simulink model "bmsTestPlatform"  (R2025b)
settings: configuration reference "cfgHarness" (kept outside this file)
PreLoadFcn:
  | if isempty(matlab.project.rootProject)
  |     % Opened outside the project (e.g. by RT-LAB): open it, then return to this folder
  |     d = pwd;
  |     try, openProject(fullfile(d, "..")); catch e, warning(e.message); end
  |     cd(d);
  | end
InitFcn:
  | plant_params
  | sensor_params
  | load_params
undefined symbols (not defined in the file): ADV_tStale, ARB_socTol, batMod, battery_builder_rtmsupport, BMS_state, BMS_stubOut, CAN_Ts, DiscIntNeverNeededParam, f, gcbh, HW_nvm, HW_powerPress, HW_resetPress, HW_rtcStart, LOAD_cycleA, LOAD_cycleAext, LOAD_iConst, LOAD_iPulse, LOAD_profile, LOAD_pulseDuty, LOAD_pulsePeriod, LOAD_scale, PLANT_switchFault, PLANT_tAmbient, PLANT_tContactor, PLANT_Ts, sens, SENS_faultChannel, SENS_faultDuration, SENS_faultRamp, SENS_faultStart, SENS_faultType, SENS_faultValue, SOC0, T0
libraries: bat_13S7P_detailed_lib x7, fl_lib x5, nesl_utility x4, simulink x3, instrumentlib x2
(part 1 of 2)
settings Model: DataDictionary=bmsPlatform.sldd  Creator=SC-Br  LastModifiedBy=SC-Br
settings ConfigSetRef: SourceName=cfgHarness

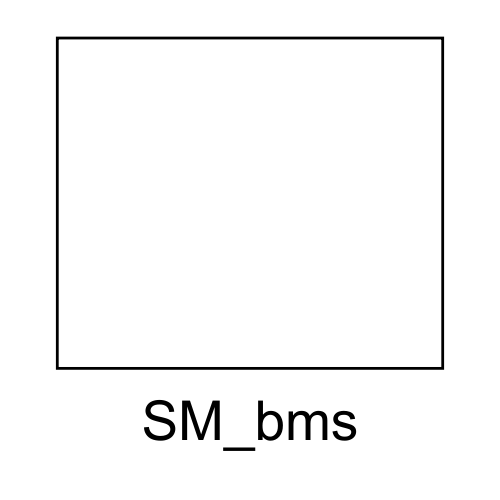
[thumbnail: Simulink's stored preview of the top-level diagram]
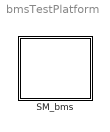
== system bmsTestPlatform ==
  SM_bms : Subsystem

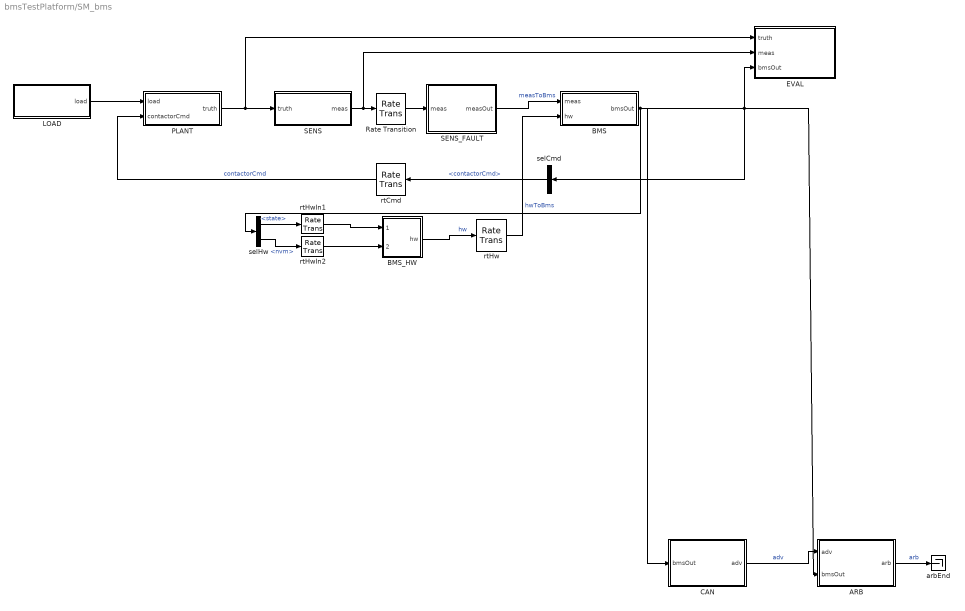
== system bmsTestPlatform/SM_bms ==
  ARB : Subsystem
  BMS : Subsystem  Variant=on  VariantControlMode=label  LabelModeActiveChoice=SIL
  BMS_HW : Subsystem
  CAN : Subsystem  Variant=on
  EVAL : Subsystem
  LOAD : Subsystem
  PLANT : Subsystem
  Rate Transition : RateTransition  Deterministic=off  OutPortSampleTimeOpt=Inherit  OutPortSampleTime=0.1
  SENS : Subsystem
  SENS_FAULT : Subsystem
  arbEnd : Terminator
  rtCmd : RateTransition  OutPortSampleTime=PLANT_Ts
  rtHw : RateTransition  Deterministic=off  OutPortSampleTimeOpt=Inherit
  rtHwIn1 : RateTransition  InitialCondition=BMS_state.OFF  OutPortSampleTime=PLANT_Ts
  rtHwIn2 : RateTransition  OutPortSampleTime=PLANT_Ts
  selCmd : BusSelector  OutputSignals=contactorCmd
  selHw : BusSelector  OutputSignals=state,nvm
  wires:
  PLANT/1(truth) -> EVAL/1(truth), SENS/1(truth)
  LOAD/1(load) -> PLANT/1(load)
  SENS/1(meas) -> EVAL/2(meas), Rate Transition/1
  BMS/1(bmsOut) -> selCmd/1, EVAL/3(bmsOut), selHw/1, CAN/1(bmsOut), ARB/2(bmsOut)
  selCmd/1 -> rtCmd/1  "<contactorCmd>"
  rtCmd/1 -> PLANT/2(contactorCmd)  "contactorCmd"
  Rate Transition/1 -> SENS_FAULT/1(meas)
  SENS_FAULT/1(measOut) -> BMS/1(meas)  "measToBms"
  BMS_HW/1(hw) -> rtHw/1  "hw"
  rtHw/1 -> BMS/2(hw)  "hwToBms"
  selHw/1 -> rtHwIn1/1  "<state>"
  rtHwIn1/1 -> BMS_HW/1(bmsState)
  selHw/2 -> rtHwIn2/1  "<nvm>"
  rtHwIn2/1 -> BMS_HW/2(nvmSaved)
  CAN/1(adv) -> ARB/1(adv)  "adv"
  ARB/1(arb) -> arbEnd/1  "arb"

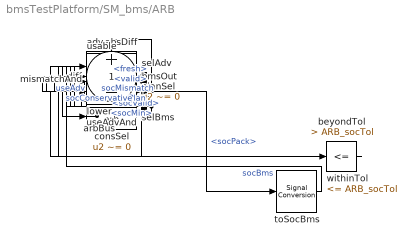
== system bmsTestPlatform/SM_bms/ARB ==
  adv : Inport
  bmsOut : Inport  Port=2
  absDiff : Abs
  arbBus : BusCreator  Inputs=5  OutDataTypeStr=Bus: ARB_bus  NonVirtualBus=on
  beyondTol : simulink/Logic and Bit Operations/Compare To Constant  relop=>  const=ARB_socTol  OutDataTypeStr=boolean
  consSel : Switch  Criteria=u2 ~= 0
  diff : Sum  Inputs=+-
  lower : MinMax  Inputs=2
  mismatchAnd : Logic
  planSel : Switch  Criteria=u2 ~= 0
  selAdv : BusSelector  OutputSignals=fresh,valid,socValid,socMin
  selBms : BusSelector  OutputSignals=socPack
  toSocBms : SignalConversion  OverrideOpt=off
  usable : Logic  Inputs=3
  useAdvAnd : Logic
  withinTol : simulink/Logic and Bit Operations/Compare To Constant  relop=<=  const=ARB_socTol  OutDataTypeStr=boolean
  arb : Outport
  wires:
  adv/1 -> selAdv/1
  bmsOut/1 -> selBms/1
  selAdv/4 -> diff/1, planSel/1, lower/1  "<socMin>"
  selBms/1 -> diff/2, planSel/3, lower/2, consSel/3, toSocBms/1  "<socPack>"
  diff/1 -> absDiff/1
  absDiff/1 -> withinTol/1, beyondTol/1
  selAdv/1 -> usable/1  "<fresh>"
  selAdv/2 -> usable/2  "<valid>"
  selAdv/3 -> usable/3  "<socValid>"
  usable/1 -> useAdvAnd/1, mismatchAnd/1, consSel/2
  withinTol/1 -> useAdvAnd/2
  beyondTol/1 -> mismatchAnd/2
  useAdvAnd/1 -> planSel/2, arbBus/1  "useAdv"
  lower/1 -> consSel/1
  mismatchAnd/1 -> arbBus/2  "socMismatch"
  planSel/1 -> arbBus/3  "socPlan"
  consSel/1 -> arbBus/4  "socConservative"
  arbBus/1 -> arb/1
  toSocBms/1 -> arbBus/5  "socBms"

== system bmsTestPlatform/SM_bms/BMS ==
  meas : Inport  OutDataTypeStr=Bus: SENS_measBus
  hw : Inport  Port=2
  SIL : ModelReference  ModelNameDialog=bms  SimulationMode=Normal  VariantControl=SIL  ModelReferenceVersion=1.43
  STUB : Subsystem  VariantControl=STUB
  bmsOut : Outport  OutDataTypeStr=Bus: BMS_outBus

== system bmsTestPlatform/SM_bms/BMS_HW ==
  note: BMS_HW - BMS board peripherals seen by the BMS (PLATFORM: stands in for the Pi's hardware; logic hwEmulator.m)
      |   OUT hw (BMS_hwIn): rtcNow = HW_rtcStart + run time (battery-backed real-time clock, s)
      |      nvm = non-volatile memory: HW_nvm at the start; replaced by the BMS's record each time it switches off
      |      powerBtn / resetBtn = button presses HW_powerPress / HW_resetPress, rows [start duration] s
      |   IN bmsState, nvmSaved: from the BMS output (one BMS step late), to store the record at switch-off
  bmsState : Inport  OutDataTypeStr=Enum: BMS_state
  nvmSaved : Inport  Port=2  OutDataTypeStr=Bus: BMS_nvmRecord
  hwFcn : MATLAB Function  TreatAsAtomicUnit=on
  runTime : DigitalClock  SampleTime=PLANT_Ts
  hw : Outport
  wires:
  runTime/1 -> hwFcn/1(t)
  bmsState/1 -> hwFcn/2(bmsState)
  nvmSaved/1 -> hwFcn/3(nvmSaved)
  hwFcn/1(hw) -> hw/1  "hw"

== system bmsTestPlatform/SM_bms/CAN ==
  note: 1) Add Subsystem or Model blocks as valid variant choices.
      | 2) You cannot connect blocks at this level. At simulation, connectivity is automatically
      | determined, based on the active variant and port name matching.
  bmsOut : Inport
  NONE : Subsystem  VariantControl=CAN_link == 0
  Subsystem1 : Subsystem  VariantControl=false
  UDP : Subsystem  VariantControl=CAN_link == 1
  adv : Outport

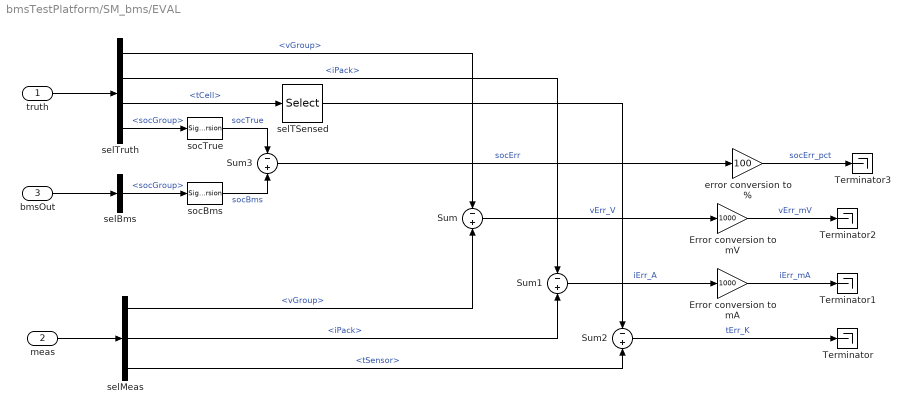
== system bmsTestPlatform/SM_bms/EVAL ==
  truth : Inport  OutDataTypeStr=Bus: PLANT_truthBus
  meas : Inport  Port=2  OutDataTypeStr=Bus: SENS_measBus
  bmsOut : Inport  Port=3  OutDataTypeStr=Bus: BMS_outBus
  Error conversion to mA : Gain  Gain=1000
  Error conversion to mV : Gain  Gain=1000
  Sum{,1..3} (4 alike) : Sum  Inputs=-+
  Terminator{,1..3} (4 alike) : Terminator
  error conversion to % : Gain  Gain=100
  selBms : BusSelector  OutputSignals=socGroup
  selMeas : BusSelector  OutputSignals=vGroup,iPack,tSensor
  selTSensed : Selector  InputPortWidth=91  IndexOptions=Index vector (dialog)  Indices=sens.T_index  OutputSizes=1
  selTruth : BusSelector  OutputSignals=vGroup,iPack,tCell,socGroup
  socBms : SignalConversion  OverrideOpt=on
  socTrue : SignalConversion  OverrideOpt=on
  wires:
  truth/1 -> selTruth/1
  selTruth/1 -> Sum/1  "<vGroup>"
  selTruth/2 -> Sum1/1  "<iPack>"
  selTruth/3 -> selTSensed/1  "<tCell>"
  meas/1 -> selMeas/1
  selMeas/2 -> Sum1/2  "<iPack>"
  selMeas/1 -> Sum/2  "<vGroup>"
  selTSensed/1 -> Sum2/1
  Sum/1 -> Error conversion to mV/1  "vErr_V"
  Sum1/1 -> Error conversion to mA/1  "iErr_A"
  Sum2/1 -> Terminator/1  "tErr_K"
  Error conversion to mV/1 -> Terminator2/1  "vErr_mV"
  Error conversion to mA/1 -> Terminator1/1  "iErr_mA"
  selMeas/3 -> Sum2/2  "<tSensor>"
  bmsOut/1 -> selBms/1
  selBms/1 -> socBms/1  "<socGroup>"
  selTruth/4 -> socTrue/1  "<socGroup>"
  Sum3/1 -> error conversion to %/1  "socErr"
  error conversion to %/1 -> Terminator3/1  "socErr_pct"
  socTrue/1 -> Sum3/1  "socTrue"
  socBms/1 -> Sum3/2  "socBms"

== system bmsTestPlatform/SM_bms/LOAD ==
  Bus Creator : BusCreator  Inputs=1  OutDataTypeStr=Bus: LOAD_bus
  LOAD_select : Subsystem
  load : Outport  OutDataTypeStr=Bus: LOAD_bus
  wires:
  LOAD_select/1(i) -> Bus Creator/1  "iDemand"
  Bus Creator/1 -> load/1

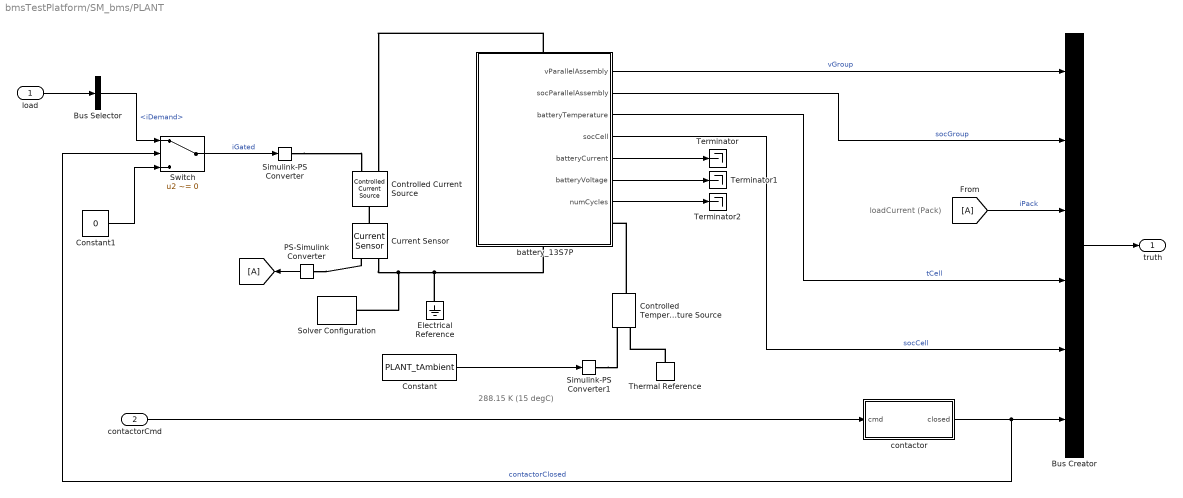
== system bmsTestPlatform/SM_bms/PLANT ==
  note: loadCurrent (Pack)
  note: 288.15 K (15 degC)
  load : Inport  OutDataTypeStr=Bus: LOAD_bus
  contactorCmd : Inport  Port=2  OutDataTypeStr=boolean
  " " : Goto
  Bus Creator : BusCreator  Inputs=6  OutDataTypeStr=Bus: PLANT_truthBus
  Bus Selector : BusSelector  OutputSignals=iDemand
  Constant : Constant  Value=PLANT_tAmbient  SampleTime=0.01
  Constant1 : Constant  Value=0
  Controlled Temperature Source : fl_lib/Thermal/Thermal Sources/Controlled Temperature Source
  Controlled Current Source : fl_lib/Electrical/Electrical Sources/Controlled Current Source
  Current Sensor : fl_lib/Electrical/Electrical Sensors/Current Sensor
  Electrical Reference : fl_lib/Electrical/Electrical Elements/Electrical Reference
  From : From
  PS-Simulink Converter : nesl_utility/PS-Simulink Converter  PhysicalDomain=network_engine_domain  SubClassName=ps_output  LeftPortType=input  RightPortType=output  PseudoPeriodic=off  Frequencies=[]  VectorFormat=inherit  Unit=inherit  AffineConversion=off
  Simulink-PS Converter : nesl_utility/Simulink-PS Converter  PhysicalDomain=network_engine_domain  SubClassName=ps_input  LeftPortType=input  RightPortType=output  PseudoPeriodic=off  Frequencies=[]  NoiseDistribution=none  NoiseParameters=[]  Unit=A  AffineConversion=off  FilteringAndDerivatives=provide  SimscapeFilterOrder=1  InputFilterTimeConstant=0.001  UdotUserProvided=0
  Simulink-PS Converter1 : nesl_utility/Simulink-PS Converter  PhysicalDomain=network_engine_domain  SubClassName=ps_input  LeftPortType=input  RightPortType=output  PseudoPeriodic=off  Frequencies=[]  NoiseDistribution=none  NoiseParameters=[]  Unit=K  AffineConversion=on  FilteringAndDerivatives=provide  SimscapeFilterOrder=1  InputFilterTimeConstant=0.001  UdotUserProvided=0
  Solver Configuration : nesl_utility/Solver Configuration  PhysicalDomain=network_engine_domain  SubClassName=solver  LeftPortType=input  RightPortType=generic  Tones=[]  Harmonics=[]  SimulateNoise=off  Profile=off  UseLocalSampling=off  EnableSwitchedLinearOptims=on  FrequencyDomain=off  UseCCode=off  RelTol=0.001  AbsTol=0.001  MinStep=1e-09  ToWorkspace=off  RevertToSquareIcSolve=off  NumHomotopyIterations=100  PhasorMode=off  PhasorModeNumHarmonics=1  ConsistencySolver=NEWTON_XTOL_AFTER_FTOL  IndexReductionMethod=DerivativeReplacement  DoDC=off  ResidualTolerance=1e-09  ConsistencyTolSource=GLOBAL  ConsistencyAbsTol=0.001  ConsistencyRelTol=0.001  ConsistencyTolFactor=0.001  UseLocalSolver=on  LocalSolverChoice=NE_BACKWARD_EULER_ADVANCER  ResolveIndetEquations=on  FunctionEvalNumThread=1  LocalSolverSampleTime=0.01  DoFixedCost=on  MaxNonlinIter=3  MaxModeIter=2  ComputeImpulses=off  ImpulseIterations=2  LinearAlgebra=auto  LinearAlgebraNumThread=0  EquationFormulation=NE_TIME_EF  DelaysMemoryBudget=1024  AutomaticFiltering=on  FilteringTimeConstant=0.001  PartitionStorageMethod=AS_NEEDED  PartitionMemoryBudget=1024  PartitionMethod=ROBUST  MultibodyUseLocalSolver=off  MultibodyLocalSolverChoice=ODE1  MultibodyLocalSolverSampleTime=0.001
  Switch : Switch  Criteria=u2 ~= 0  SaturateOnIntegerOverflow=off  InputSameDT=off
  Terminator : Terminator
  Terminator1 : Terminator
  Terminator2 : Terminator
  Thermal Reference : fl_lib/Thermal/Thermal Elements/Thermal Reference
  battery_13S7P : Subsystem  LoadFcn=battery_builder_rtmsupport('loadfcn',gcbh);
      settings: CopyFcn=battery_builder_rtmsupport('copyfcn',gcbh);  PreCopyFcn=battery_builder_rtmsupport('precopyfcn',gcbh);  PreDeleteFcn=battery_builder_rtmsupport('predeletefcn',gcbh);  PortSchema="{\"entries\":[{\"content\":{\"sides\":[{\"content\":{\"connectorIds\":[\"LConn1\"]},\"type\":\"ConnectorPlacement.EquallySpacedRectSide\",\"uuid\":\"2e680de8-6342-42e2-9168-c81c1b12a645\"},{\"content\":{\"connectorIds\":[\"RConn1\"],\"side\":\"RIGHT\"},\"type\":\"ConnectorPlacement.EquallySpacedRectSide\",\"uuid\":\"bd266347-41ea-4c6d-a3ed-ea2dbc6fb3bf\"},{\"content\":{\"side\":\"TOP\"},\"type\":\"ConnectorPlacement.EquallySpacedRectSide\",\"uuid\":\"bb482786-eee9-47ff-b272-bd5b61deceb7\"},{\"content\":{\"connectorIds\":[\"Out1\",\"Out2\",\"Out3\",\"Out4\",\"Out5\",\"Out6\",\"Out7\",\"RConn2\"],\"side\":\"BOTTOM\"},\"type\":\"ConnectorPlacement.EquallySpacedRectSide\",\"uuid\":\"55ff33fa-2818-4bd8-9314-362004ddf12e\"}]},\"type\":\"ConnectorPlacement.EquallySpacedConnector\",\"uuid\":\"a7cd390e-be11-454d-a765-ee13c925b2c2\"}],\"packageUris\":[\"http://schema.mathworks.com/mf0/Connector/R2020b\"],\"version\":\"1.0\"}"
      mask Display: image('batteryImage.png');
  contactor : Subsystem  TreatAsAtomicUnit=on
  truth : Outport  OutDataTypeStr=Bus: PLANT_truthBus
  wires:
  load/1 -> Bus Selector/1
  Bus Selector/1 -> Switch/1  "<iDemand>"
  battery_13S7P/1(vParallelAssembly) -> Bus Creator/1  "vGroup"
  battery_13S7P/2(socParallelAssembly) -> Bus Creator/2  "socGroup"
  battery_13S7P/3(batteryTemperature) -> Bus Creator/4  "tCell"
  battery_13S7P/4(socCell) -> Bus Creator/5  "socCell"
  PS-Simulink Converter/1 -> " "/1
  From/1 -> Bus Creator/3  "iPack"
  battery_13S7P/5(batteryCurrent) -> Terminator/1
  battery_13S7P/6(batteryVoltage) -> Terminator1/1
  battery_13S7P/7(numCycles) -> Terminator2/1
  Bus Creator/1 -> truth/1
  Constant/1 -> Simulink-PS Converter1/1
  Constant1/1 -> Switch/3
  Switch/1 -> Simulink-PS Converter/1  "iGated"
  contactorCmd/1 -> contactor/1(cmd)
  contactor/1(closed) -> Switch/2, Bus Creator/6  "contactorClosed"
  connections:
  battery_13S7P/LConn1 -- Controlled Current Source/RConn2
  battery_13S7P/RConn1 -- Solver Configuration/RConn1 -- Current Sensor/RConn2 -- Electrical Reference/LConn1
  Simulink-PS Converter/RConn1 -- Controlled Current Source/RConn1
  Current Sensor/LConn1 -- Controlled Current Source/LConn1
  Controlled Temperature Source/LConn1 -- battery_13S7P/RConn2
  Thermal Reference/LConn1 -- Controlled Temperature Source/RConn2
  Simulink-PS Converter1/RConn1 -- Controlled Temperature Source/RConn1
  PS-Simulink Converter/LConn1 -- Current Sensor/RConn1

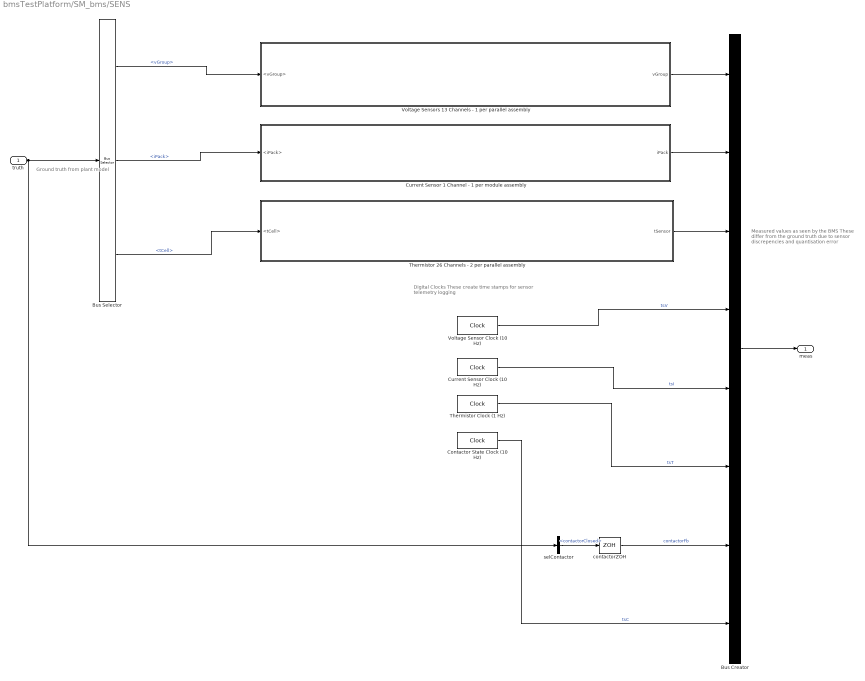
== system bmsTestPlatform/SM_bms/SENS ==
  note: Ground truth from
      | plant model
  note: Digital Clocks
      |
      | These create time stamps for sensor telemetry logging
  note: Measured values as
      | seen by the BMS
      |
      | These differ from the ground truth due to
      | sensor discrepencies and quantisation error
  truth : Inport  OutDataTypeStr=Bus: PLANT_truthBus
  " Thermistor Clock (1 Hz)" : DigitalClock  SampleTime=sens.Ts_T
  Bus Creator : BusCreator  Inputs=8  OutDataTypeStr=Bus: SENS_measBus
  Bus Selector : BusSelector  OutputSignals=vGroup,iPack,tCell
  Contactor State Clock (10 Hz) : DigitalClock  SampleTime=sens.Ts_C
  Current Sensor 1 Channel - 1 per module assembly : Subsystem
  Current Sensor Clock (10 Hz) : DigitalClock  SampleTime=sens.Ts_I
  Thermistor 26 Channels - 2 per parallel assembly : Subsystem
  Voltage Sensor Clock (10 Hz) : DigitalClock  SampleTime=sens.Ts_V
  Voltage Sensors 13 Channels - 1 per parallel assembly : Subsystem
  contactorZOH : ZeroOrderHold  SampleTime=sens.Ts_C
  selContactor : BusSelector  OutputSignals=contactorClosed
  meas : Outport  OutDataTypeStr=Bus: SENS_measBus
  wires:
  truth/1 -> Bus Selector/1, selContactor/1
  Bus Creator/1 -> meas/1
  Bus Selector/1 -> Voltage Sensors 13 Channels - 1 per parallel assembly/1(<vGroup>)  "<vGroup>"
  Voltage Sensors 13 Channels - 1 per parallel assembly/1(vGroup) -> Bus Creator/1
  Bus Selector/2 -> Current Sensor 1 Channel - 1 per module assembly/1(<iPack>)  "<iPack>"
  Current Sensor 1 Channel - 1 per module assembly/1(iPack) -> Bus Creator/2
  Bus Selector/3 -> Thermistor 26 Channels - 2 per parallel assembly/1(<tCell>)  "<tCell>"
  Voltage Sensor Clock (10 Hz)/1 -> Bus Creator/4  "tsV"
  Current Sensor Clock (10 Hz)/1 -> Bus Creator/5  "tsI"
  " Thermistor Clock (1 Hz)"/1 -> Bus Creator/6  "tsT"
  Thermistor 26 Channels - 2 per parallel assembly/1(tSensor) -> Bus Creator/3
  selContactor/1 -> contactorZOH/1  "<contactorClosed>"
  contactorZOH/1 -> Bus Creator/7  "contactorFb"
  Contactor State Clock (10 Hz)/1 -> Bus Creator/8  "tsC"

== system bmsTestPlatform/SM_bms/SENS_FAULT ==
  note: SENS_FAULT - measurement fault injection (PLATFORM ONLY, never part of the BMS)
      |   In/Out: SENS_measBus at the BMS rate. Logic in sensFaultInject.m
      |   SENS_faultType: 0 none | 1 voltage offset | 2 temperature offset | 3 temperatures stop updating | 4 voltage channel open
      |   SENS_faultChannel: group 1-13 or sensor 1-26 | SENS_faultValue: offset (V or K)
      |   SENS_faultStart / SENS_faultDuration / SENS_faultRamp (s): when, how long, ramp-in time
  meas : Inport  OutDataTypeStr=Bus: SENS_measBus
  faultFcn : MATLAB Function  TreatAsAtomicUnit=on
  measOut : Outport
  wires:
  meas/1 -> faultFcn/1(m)
  faultFcn/1(mOut) -> measOut/1

== system bmsTestPlatform/SM_bms/BMS/STUB ==
  meas : Inport
  hw : Inport  Port=2
  Terminator : Terminator
  TerminatorHw : Terminator
  bmsOutStub : Constant  Value=BMS_stubOut  OutDataTypeStr=Bus: BMS_outBus
  bmsOut : Outport
  wires:
  meas/1 -> Terminator/1
  bmsOutStub/1 -> bmsOut/1
  hw/1 -> TerminatorHw/1

== system bmsTestPlatform/SM_bms/CAN/NONE ==
  bmsOut : Inport
  advStub : MATLAB Function  TreatAsAtomicUnit=on
  unused : Terminator
  adv : Outport
  wires:
  bmsOut/1 -> unused/1
  advStub/1(adv) -> adv/1

== system bmsTestPlatform/SM_bms/CAN/Subsystem1 ==
  bmsOut : Inport
  adv : Outport

== system bmsTestPlatform/SM_bms/CAN/UDP ==
  bmsOut : Inport
  canRx : MATLAB Function  TreatAsAtomicUnit=on
  canTx : MATLAB Function  TreatAsAtomicUnit=on
  udpReceive : instrumentlib/UDP Receive  LocalAddress=0.0.0.0  LocalPort=50001  EnablePortSharing=off  Host=192.168.50.2  Port=50000  GetLatestData=on  DataSize=[128 1]  DataType=uint8  ASCIIFormatting=%f,  Terminator=LF  CustomTerminator=10  ByteOrder=big-endian  EnableBlockingMode=off  Timeout=10  SampleTime=CAN_Ts  SimulateUsing=Interpreted execution
  udpSend : instrumentlib/UDP Send  Host=192.168.50.2  Port=50000  LocalAddress=0.0.0.0  LocalPort=-1  EnablePortSharing=off  OutputDatagramPacketSize=512  ByteOrder=big-endian  EnableBlockingMode=on  SimulateUsing=Interpreted execution
  adv : Outport
  wires:
  bmsOut/1 -> canTx/1(b)
  canTx/1(frames) -> udpSend/1
  udpReceive/1 -> canRx/1(data)
  udpReceive/2 -> canRx/2(status)
  canRx/1(adv) -> adv/1

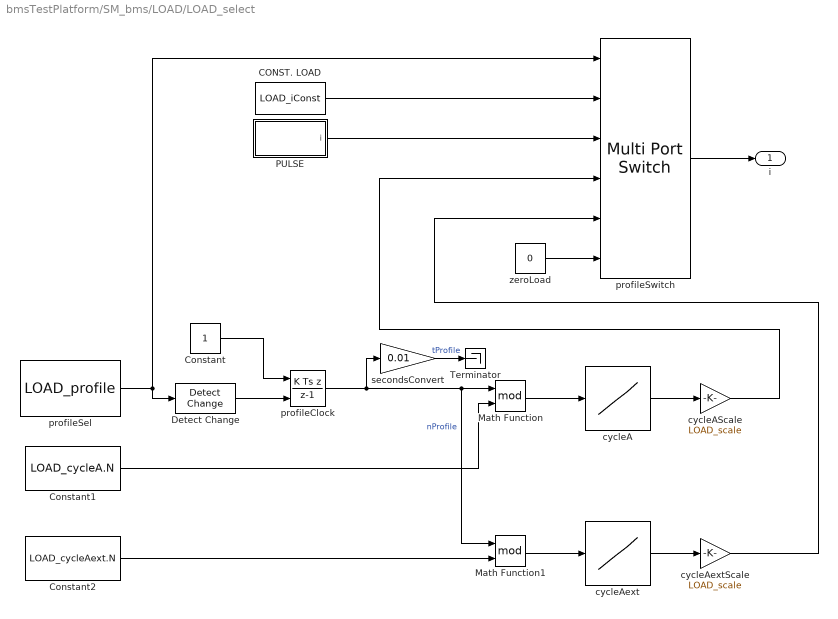
== system bmsTestPlatform/SM_bms/LOAD/LOAD_select ==
  CONST. LOAD : Constant  Value=LOAD_iConst  SampleTime=0.01
  Constant : Constant  SampleTime=0.01
  Constant1 : Constant  Value=LOAD_cycleA.N
  Constant2 : Constant  Value=LOAD_cycleAext.N
  Detect Change : simulink/Logic and Bit Operations/Detect Change  vinit=0  OutDataTypeStr=boolean
  Math Function : Math  Operator=mod
  Math Function1 : Math  Operator=mod
  PULSE : Subsystem  VariantControl=LOAD_variant == 2
  Terminator : Terminator
  cycleA : Lookup_n-D  NumberOfTableDimensions=1  BreakpointsSpecification=Even spacing  BreakpointsForDimension1=[-5:5]  BreakpointsForDimension1FirstPoint=0  BreakpointsForDimension1Spacing=LOAD_cycleA.k  Table=LOAD_cycleA.i  InterpMethod=Flat  InternalRulePriority=Speed  RndMeth=Simplest
  cycleAScale : Gain  Gain=LOAD_scale
  cycleAext : Lookup_n-D  NumberOfTableDimensions=1  BreakpointsSpecification=Even spacing  BreakpointsForDimension1=[-5:5]  BreakpointsForDimension1FirstPoint=0  BreakpointsForDimension1Spacing=LOAD_cycleAext.k  Table=LOAD_cycleAext.i  InterpMethod=Flat  InternalRulePriority=Speed  RndMeth=Simplest
  cycleAextScale : Gain  Gain=LOAD_scale
  profileClock : DiscreteIntegrator  IntegratorMethod=Integration: Backward Euler  gainval=100  ExternalReset=level  SampleTime=0.01  ICPrevOutput=DiscIntNeverNeededParam  ICPrevScaledInput=DiscIntNeverNeededParam
  profileSel : Constant  Value=LOAD_profile  SampleTime=0.01
  profileSwitch : MultiPortSwitch  Inputs=4  DataPortForDefault=Additional data port  DiagnosticForDefault=None  SaturateOnIntegerOverflow=off  InputSameDT=off
  secondsConvert : Gain  Gain=0.01
  zeroLoad : Constant  Value=0
  i : Outport
  wires:
  profileSel/1 -> profileSwitch/1, Detect Change/1
  Constant/1 -> profileClock/1
  Detect Change/1 -> profileClock/2
  Constant1/1 -> Math Function/2
  Constant2/1 -> Math Function1/2
  Math Function/1 -> cycleA/1
  Math Function1/1 -> cycleAext/1
  cycleA/1 -> cycleAScale/1
  cycleAext/1 -> cycleAextScale/1
  profileSwitch/1 -> i/1
  CONST. LOAD/1 -> profileSwitch/2
  PULSE/1(i) -> profileSwitch/3
  cycleAScale/1 -> profileSwitch/4
  cycleAextScale/1 -> profileSwitch/5
  zeroLoad/1 -> profileSwitch/6
  profileClock/1 -> secondsConvert/1, Math Function1/1, Math Function/1  "nProfile"
  secondsConvert/1 -> Terminator/1  "tProfile"

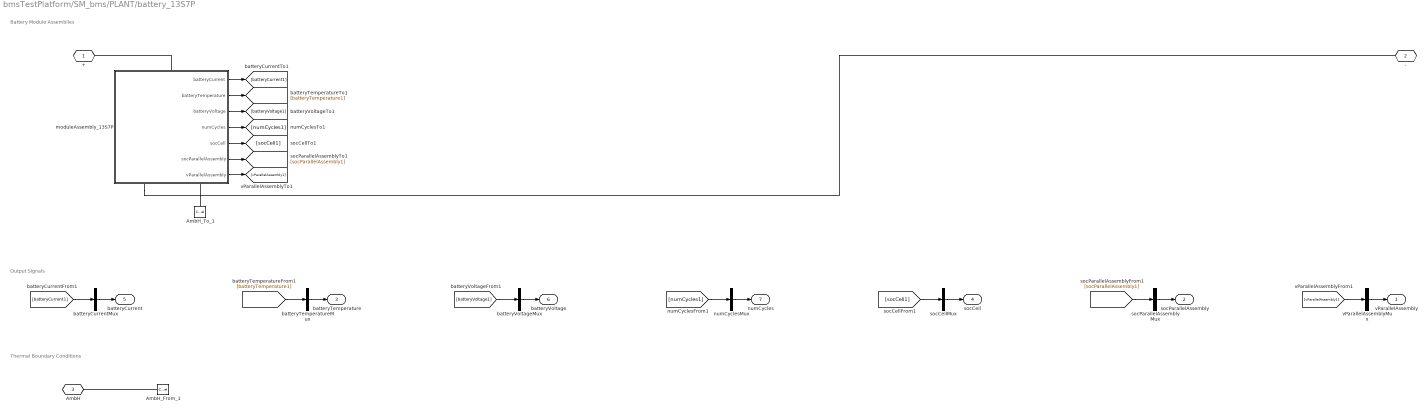
== system bmsTestPlatform/SM_bms/PLANT/battery_13S7P ==
  note: Battery Module Assemblies
  note: Output Signals
  note: Thermal Boundary Conditions
  AmbH_From_1 : ConnectionLabel  Label=ambH_1
  AmbH_To_1 : ConnectionLabel  Label=ambH_1
  batteryCurrentMux : Mux  Inputs=1
  batteryTemperatureMux : Mux  Inputs=1
  batteryVoltageMux : Mux  Inputs=1
  moduleAssembly_13S7P : Subsystem  LoadFcn=battery_builder_rtmsupport('loadfcn',gcbh);
      settings: CopyFcn=battery_builder_rtmsupport('copyfcn',gcbh);  PreCopyFcn=battery_builder_rtmsupport('precopyfcn',gcbh);  PreDeleteFcn=battery_builder_rtmsupport('predeletefcn',gcbh);  PortSchema="{\"entries\":[{\"content\":{\"sides\":[{\"content\":{\"connectorIds\":[\"LConn1\"]},\"type\":\"ConnectorPlacement.EquallySpacedRectSide\",\"uuid\":\"2e680de8-6342-42e2-9168-c81c1b12a645\"},{\"content\":{\"connectorIds\":[\"RConn1\",\"RConn2\"],\"side\":\"RIGHT\"},\"type\":\"ConnectorPlacement.EquallySpacedRectSide\",\"uuid\":\"bd266347-41ea-4c6d-a3ed-ea2dbc6fb3bf\"},{\"content\":{\"side\":\"TOP\"},\"type\":\"ConnectorPlacement.EquallySpacedRectSide\",\"uuid\":\"bb482786-eee9-47ff-b272-bd5b61deceb7\"},{\"content\":{\"connectorIds\":[\"Out1\",\"Out2\",\"Out3\",\"Out4\",\"Out5\",\"Out6\",\"Out7\"],\"side\":\"BOTTOM\"},\"type\":\"ConnectorPlacement.EquallySpacedRectSide\",\"uuid\":\"56f55342-be9c-46ac-b4cc-a736fce22cf1\"}]},\"type\":\"ConnectorPlacement.EquallySpacedConnector\",\"uuid\":\"a7cd390e-be11-454d-a765-ee13c925b2c2\"}],\"packageUris\":[\"http://schema.mathworks.com/mf0/Connector/R2020b\"],\"version\":\"1.0\"}"
      mask Display: image('$imagefile')
  numCyclesMux : Mux  Inputs=1
  socCellMux : Mux  Inputs=1
  socParallelAssemblyMux : Mux  Inputs=1
  vParallelAssemblyMux : Mux  Inputs=1
  + : PMIOPort  Side=Left
  - : PMIOPort  Port=2  Side=Right
  AmbH : PMIOPort  Port=3  Side=Right  ConnectionType=Connection: foundation.thermal.thermal
  vParallelAssembly : Outport
  socParallelAssembly : Outport  Port=2
  batteryTemperature : Outport  Port=3
  socCell : Outport  Port=4
  batteryCurrent : Outport  Port=5
  batteryVoltage : Outport  Port=6
  numCycles : Outport  Port=7
  wires:
  moduleAssembly_13S7P/1(batteryCurrent) -> [batteryCurrent1]
  batteryCurrentMux/1 -> batteryCurrent/1
  [batteryCurrent1] -> batteryCurrentMux/1
  moduleAssembly_13S7P/2(batteryTemperature) -> [batteryTemperature1]
  batteryTemperatureMux/1 -> batteryTemperature/1
  [batteryTemperature1] -> batteryTemperatureMux/1
  moduleAssembly_13S7P/3(batteryVoltage) -> [batteryVoltage1]
  batteryVoltageMux/1 -> batteryVoltage/1
  [batteryVoltage1] -> batteryVoltageMux/1
  moduleAssembly_13S7P/4(numCycles) -> [numCycles1]
  numCyclesMux/1 -> numCycles/1
  [numCycles1] -> numCyclesMux/1
  moduleAssembly_13S7P/5(socCell) -> [socCell1]
  socCellMux/1 -> socCell/1
  [socCell1] -> socCellMux/1
  moduleAssembly_13S7P/6(socParallelAssembly) -> [socParallelAssembly1]
  socParallelAssemblyMux/1 -> socParallelAssembly/1
  [socParallelAssembly1] -> socParallelAssemblyMux/1
  moduleAssembly_13S7P/7(vParallelAssembly) -> [vParallelAssembly1]
  vParallelAssemblyMux/1 -> vParallelAssembly/1
  [vParallelAssembly1] -> vParallelAssemblyMux/1
  connections:
  moduleAssembly_13S7P/LConn1 -- +/RConn1
  moduleAssembly_13S7P/RConn1 -- -/RConn1
  AmbH_To_1/LConn1 -- moduleAssembly_13S7P/RConn2
  AmbH_From_1/LConn1 -- AmbH/RConn1

== system bmsTestPlatform/SM_bms/PLANT/contactor ==
  cmd : Inport
  Delay : Delay  DelayLength=round(PLANT_tContactor/PLANT_Ts)  InitialCondition=false  SampleTime=PLANT_Ts
  faultSel : Constant  Value=PLANT_switchFault  SampleTime=PLANT_Ts
  faultSwitch : MultiPortSwitch  DataPortOrder=Zero-based contiguous  DataPortForDefault=Additional data port  DiagnosticForDefault=None  zeroidx=on  SaturateOnIntegerOverflow=off  InputSameDT=off
  stuckOpen : Constant  Value=false  OutDataTypeStr=boolean  SampleTime=PLANT_Ts
  welded : Constant  Value=true  OutDataTypeStr=boolean  SampleTime=PLANT_Ts
  closed : Outport
  wires:
  Delay/1 -> faultSwitch/5, faultSwitch/2
  faultSel/1 -> faultSwitch/1
  stuckOpen/1 -> faultSwitch/3
  welded/1 -> faultSwitch/4
  faultSwitch/1 -> closed/1
  cmd/1 -> Delay/1

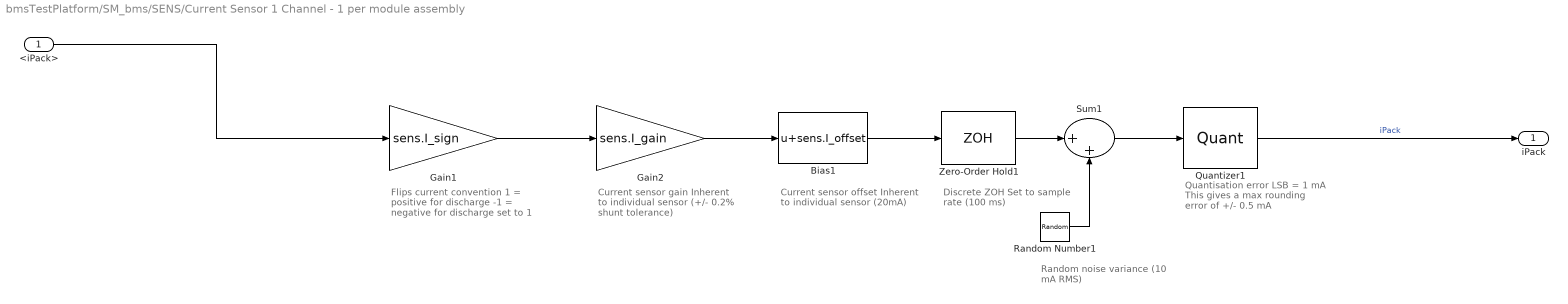
== system bmsTestPlatform/SM_bms/SENS/Current Sensor 1 Channel - 1 per module assembly ==
  note: Current sensor gain
      |
      | Inherent to individual sensor (+/- 0.2% shunt tolerance)
  note: Current sensor offset
      |
      | Inherent to individual sensor (20mA)
  note: Discrete ZOH
      |
      | Set to sample rate
      | (100 ms)
  note: Random noise
      |
      | variance (10 mA RMS)
  note: Quantisation error
      |
      | LSB = 1 mA
      |
      | This gives a max rounding
      | error of +/- 0.5 mA
  note: Flips current convention
      |
      | 1 = positive for discharge
      | -1 = negative for discharge
      |
      | set to 1
  <iPack> : Inport
  Bias1 : Bias  Bias=sens.I_offset  SaturateOnIntegerOverflow=off
  Gain1 : Gain  Gain=sens.I_sign
  Gain2 : Gain  Gain=sens.I_gain
  Quantizer1 : Quantizer  QuantizationInterval=sens.I_lsb
  Random Number1 : RandomNumber  Variance=sens.I_noiseVar  Seed=sens.I_seed  SampleTime=sens.Ts_I
  Sum1 : Sum  Inputs=|++
  Zero-Order Hold1 : ZeroOrderHold  SampleTime=sens.Ts_I
  iPack : Outport
  wires:
  Quantizer1/1 -> iPack/1  "iPack"
  <iPack>/1 -> Gain1/1
  Gain1/1 -> Gain2/1
  Gain2/1 -> Bias1/1
  Bias1/1 -> Zero-Order Hold1/1
  Zero-Order Hold1/1 -> Sum1/1
  Sum1/1 -> Quantizer1/1
  Random Number1/1 -> Sum1/2

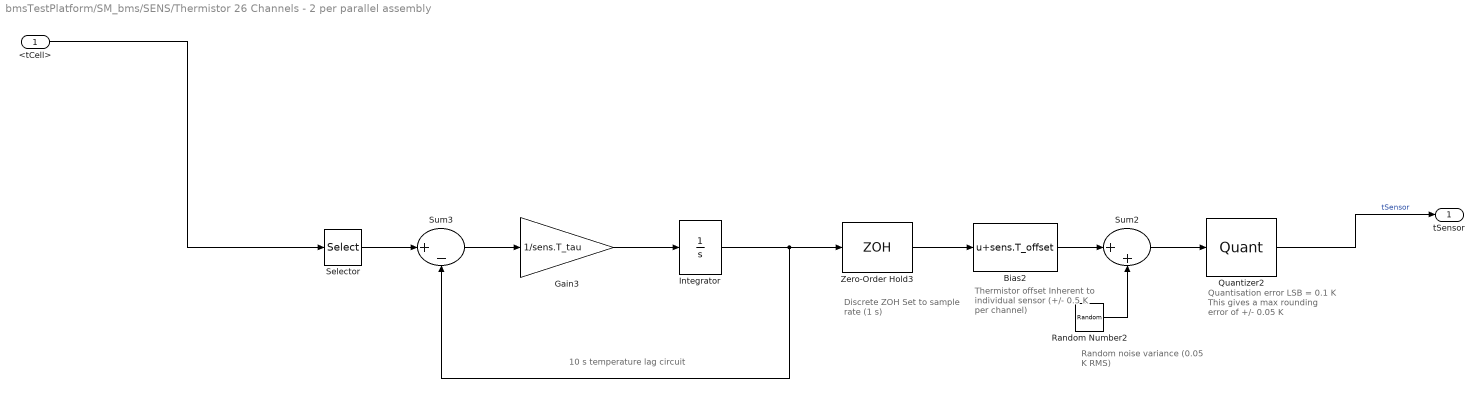
== system bmsTestPlatform/SM_bms/SENS/Thermistor 26 Channels - 2 per parallel assembly ==
  note: 10 s temperature lag circuit
  note: Discrete ZOH
      |
      | Set to sample rate
      | (1 s)
  note: Thermistor offset
      |
      | Inherent to individual sensor (+/- 0.5 K per channel)
  note: Random noise
      |
      | variance (0.05 K RMS)
  note: Quantisation error
      |
      | LSB = 0.1 K
      |
      | This gives a max rounding
      | error of +/- 0.05 K
  <tCell> : Inport
  Bias2 : Bias  Bias=sens.T_offset  SaturateOnIntegerOverflow=off
  Gain3 : Gain  Gain=1/sens.T_tau
  Integrator : Integrator  InitialCondition=T0*ones(26,1)
  Quantizer2 : Quantizer  QuantizationInterval=sens.T_lsb
  Random Number2 : RandomNumber  Variance=sens.T_noiseVar  Seed=sens.T_seed  SampleTime=sens.Ts_T
  Selector : Selector  InputPortWidth=91  IndexOptions=Index vector (dialog)  Indices=sens.T_index  OutputSizes=1  RuntimeRangeChecks=on
  Sum2 : Sum  Inputs=|++
  Sum3 : Sum  Inputs=|+-
  Zero-Order Hold3 : ZeroOrderHold  SampleTime=sens.Ts_T
  tSensor : Outport
  wires:
  Sum2/1 -> Quantizer2/1
  Random Number2/1 -> Sum2/2
  Sum3/1 -> Gain3/1
  Bias2/1 -> Sum2/1
  Integrator/1 -> Sum3/2, Zero-Order Hold3/1
  Selector/1 -> Sum3/1
  Zero-Order Hold3/1 -> Bias2/1
  Gain3/1 -> Integrator/1
  <tCell>/1 -> Selector/1
  Quantizer2/1 -> tSensor/1  "tSensor"

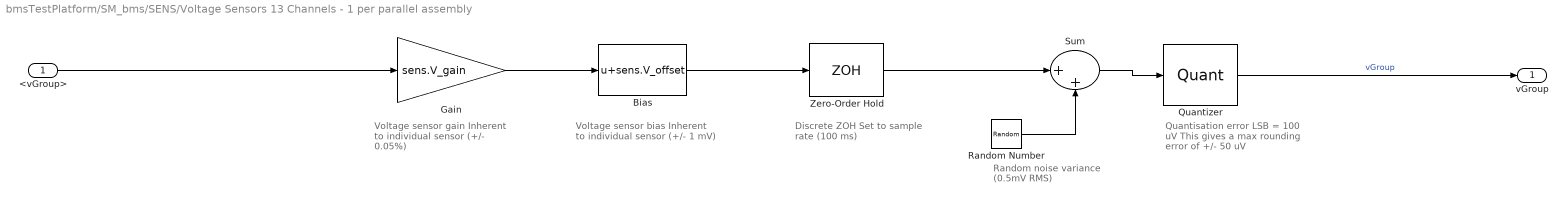
== system bmsTestPlatform/SM_bms/SENS/Voltage Sensors 13 Channels - 1 per parallel assembly ==
  note: Voltage sensor gain
      |
      | Inherent to individual sensor (+/- 0.05%)
  note: Random noise
      |
      | variance (0.5mV RMS)
  note: Voltage sensor bias
      |
      | Inherent to individual sensor
      | (+/- 1 mV)
  note: Discrete ZOH
      |
      | Set to sample rate
      | (100 ms)
  note: Quantisation error
      |
      | LSB = 100 uV
      |
      | This gives a max rounding
      | error of +/- 50 uV
  <vGroup> : Inport
  Bias : Bias  Bias=sens.V_offset  SaturateOnIntegerOverflow=off
  Gain : Gain  Gain=sens.V_gain
  Quantizer : Quantizer  QuantizationInterval=sens.V_lsb
  Random Number : RandomNumber  Variance=sens.V_noiseVar  Seed=sens.V_seed  SampleTime=sens.Ts_V
  Sum : Sum  Inputs=|++
  Zero-Order Hold : ZeroOrderHold  SampleTime=sens.Ts_V
  vGroup : Outport
  wires:
  Sum/1 -> Quantizer/1
  Gain/1 -> Bias/1
  <vGroup>/1 -> Gain/1
  Bias/1 -> Zero-Order Hold/1
  Zero-Order Hold/1 -> Sum/1
  Quantizer/1 -> vGroup/1  "vGroup"
  Random Number/1 -> Sum/2

== system bmsTestPlatform/SM_bms/LOAD/LOAD_select/PULSE ==
  Pulse Generator : DiscretePulseGenerator  PulseType=Time based  Amplitude=LOAD_iPulse  Period=LOAD_pulsePeriod  PulseWidth=LOAD_pulseDuty
  i : Outport
  wires:
  Pulse Generator/1 -> i/1
